simulink model "sid_test"  (R2025b)
settings: Solver=VariableStepAuto  StartTime=0.0  StopTime=10.0  RelTol=1e-3
values from neighbouring files (symbols this model uses):
  P = satellite_params()    [individual_test_with_dynamics.m]    (also in parameters.m; test.m = thrusters(:, 1:3))
  q_ref = [ cos(theta_ref/2) ... (first row only)    [parameters.m]
libraries: aerolibutil x2
settings Model: Creator=ADMIN  LastModifiedBy=ADMIN

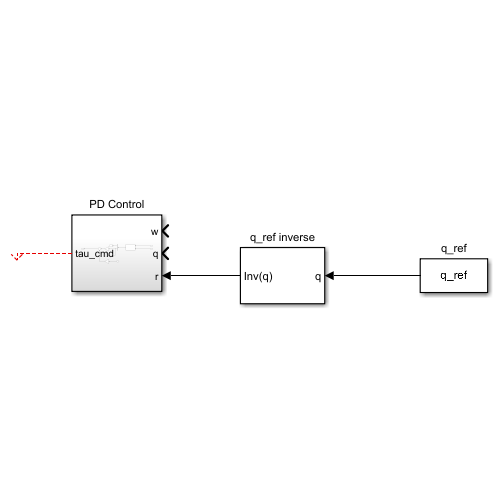
[thumbnail: Simulink's stored preview of the top-level diagram]
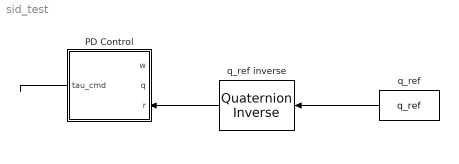
== system sid_test ==
  PD Control : Subsystem
  q_ref : Constant  Value=q_ref
  q_ref inverse : aerolibutil/Quaternion Inverse
  wires:
  q_ref inverse/1 -> PD Control/3(r)
  q_ref/1 -> q_ref inverse/1
  PD Control/1(tau_cmd) -> ?

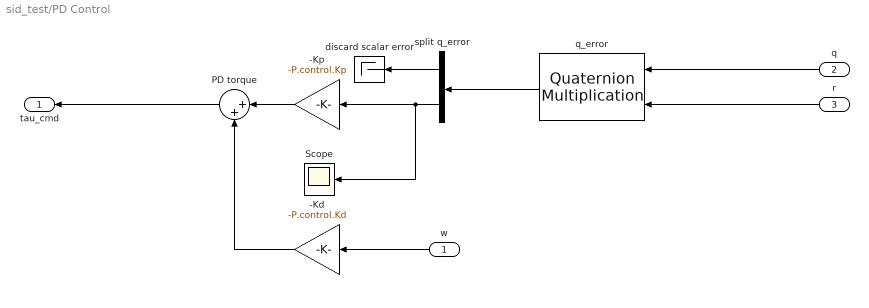
== system sid_test/PD Control ==
  w : Inport
  q : Inport  Port=2
  r : Inport  Port=3
  -Kd : Gain  Gain=-P.control.Kd
  -Kp : Gain  Gain=-P.control.Kp
  PD torque : Sum  Inputs=|++
  Scope : Scope
      settings: ActiveDisplayYMinimum=-1  ActiveDisplayYMaximum=1
  discard scalar error : Terminator
  q_error : aerolibutil/Quaternion Multiplication
  split q_error : Demux  Outputs=[1 3]
  tau_cmd : Outport
  wires:
  split q_error/2 -> -Kp/1, Scope/1
  split q_error/1 -> discard scalar error/1
  q_error/1 -> split q_error/1
  -Kp/1 -> PD torque/1
  -Kd/1 -> PD torque/2
  w/1 -> -Kd/1
  PD torque/1 -> tau_cmd/1
  q/1 -> q_error/1
  r/1 -> q_error/2
